simulink model "im_inv_sensorless_ctrl_model"  (R2026a)
settings: Solver=ode1  StopTime=simlength  FixedStep=tc  MaxStep=tc  EnableMultiTasking=on
values from neighbouring files (symbols this model uses):
  cp = 2    [im_param_calc_3.m]
  Ibez = Inom*sqrt(2)    [im_param_calc_3.m]
  Lm = Ls - Lds    [im_param_calc_3.m]
  Lr = Lm + Ldr    [im_param_calc_3.m]
  Ls = Vnom/sqrt(3)/I0/(2*pi*fnom)    [im_param_calc_3.m]
  Rr = Rr+deltaRr    (= 0.00099)    [im_param_calc_3.m]
  Rs = PhaseResistance    (= 0.009)    [im_param_calc_3.m]
undefined symbols (not defined in the file or in its folder): Adrso_im, alpha_norm, beta_norm, Crso_im, CTRPIFF_CLIP_RELEASE, dead_time, DiscIntNeverNeededParam, emf_fb_p, emf_p, fi_rot_ref_norm, fPWM_INV, gamma_norm, iq_lim, Jm_model, kg, ki_inv_d, ki_inv_q, ki_w, kp_inv_d, kp_inv_q, kp_w, kw, Ldrso_im, Lm_norm, Lr_norm, Ls_norm, magnitude, Omega_r_bez, Omega_s_bez, Rs_norm, sigma_norm, simlength, tc, Tcontrol_INV, timeRamp, Tload, ts_afe, ts_inv, uf_omega_ref, uf_uq_ref, wref
libraries: nesl_utility x64, fl_lib x49, simulink x2, im_uvw_2_lib x1, threephase_inductor_lib x1, cstblocks_lti x1
(part 3 of 4)

== system im_inv_sensorless_ctrl_model/inverter//ctrl/im_ctrl/rotor_speed_observer/pi ==
  u_ref : Inport
  u : Inport  Port=2
  1/Ti : Gain  Gain=kp  SaturateOnIntegerOverflow=on  OutDataTypeStr=Inherit: Same as input  ParamDataTypeStr=Inherit: Same as input
  Saturation : Saturate  UpperLimit=lim_up  LowerLimit=lim_down
  Sum1 : Sum  Inputs=+++  SaturateOnIntegerOverflow=on
  Sum2 : Sum  Inputs=-+  SaturateOnIntegerOverflow=on
  Sum3 : Sum  Inputs=-+  SaturateOnIntegerOverflow=on
  Unit Delay4 : UnitDelay  SampleTime=-1
  kp : Gain  Gain=ki  SaturateOnIntegerOverflow=on  OutDataTypeStr=Inherit: Same as input  ParamDataTypeStr=Inherit: Same as input
  y : Outport
  wires:
  1/Ti/1 -> Sum1/1, Sum3/1
  kp/1 -> Sum1/2
  Sum3/1 -> Unit Delay4/1
  Unit Delay4/1 -> Sum1/3
  u_ref/1 -> Sum2/2
  u/1 -> Sum2/1
  Sum2/1 -> kp/1, 1/Ti/1
  Sum1/1 -> Saturation/1
  Saturation/1 -> Sum3/2, y/1

== system im_inv_sensorless_ctrl_model/inverter//ctrl/im_ctrl/rotor_speed_observer/voltage_flux_estimator ==
  Gain : Gain
  Gain1 : Gain
  Trigonometric Function : Trigonometry  Operator=cos
  Trigonometric Function1 : Trigonometry
  Zero-Order Hold{,1..3} (4 alike) : ZeroOrderHold  SampleTime=ts_inv
  flux_observers_from_voltage_model : Scope  NumInputPorts=2
      settings: ActiveDisplayYMinimum=-0.67163437881991128  ActiveDisplayYMaximum=0.85448846422944114  DataLoggingVariableName=ScopeData4
  psi_alpha_hat : Subsystem
  psi_beta_hat : Subsystem
  tag scope: psi_r_alpha_vhat_mod1=global, psi_r_beta_vhat_mod1=global, psi_r_m_alpha=global, psi_r_m_beta=global
  wires:
  Zero-Order Hold3/1 -> psi_beta_hat/2(ibeta)
  psi_alpha_hat/1(psi_r_alpha_hat) -> [psi_r_alpha_vhat_mod1]
  [is_alpha_pu_mod1] -> Zero-Order Hold2/1
  [uctrl_alpha_mod1] -> Zero-Order Hold/1
  [is_beta_pu_mod1] -> Zero-Order Hold3/1
  psi_beta_hat/1(psi_r_beta_hat) -> [psi_r_beta_vhat_mod1]
  [uctrl_beta_mod1] -> Zero-Order Hold1/1
  Zero-Order Hold2/1 -> psi_alpha_hat/2(ialpha)
  Zero-Order Hold/1 -> psi_alpha_hat/1(ualpha)
  Zero-Order Hold1/1 -> psi_beta_hat/1(ubeta)
  [theta_s_mod1] -> Trigonometric Function/1, Trigonometric Function1/1
  Trigonometric Function/1 -> Gain/1
  Trigonometric Function1/1 -> Gain1/1
  Gain1/1 -> [psi_r_m_beta]
  Gain/1 -> [psi_r_m_alpha]
  [psi_r_alpha_vhat_mod1] -> flux_observers_from_voltage_model/1
  [psi_r_beta_vhat_mod1] -> flux_observers_from_voltage_model/2

== system im_inv_sensorless_ctrl_model/inverter//ctrl/inverter/inverter/sv_pwm ==
  ab : Inport
  enable : Inport  Port=2
  pwm_phase : Inport  Port=3
  -1<x<1 : Saturate  UpperLimit=1  LowerLimit=-1
  Bus Selector : BusSelector  OutputSignals=da,db,dc
  C Caller : CCaller  FunctionName=sv_pwm_process_simulink  PortSpecificationStruct="%)30     .    V @   8    (     @         %    \"     4    !     0         %  0 \"0    $    _    07)G3F%M90  4&]R=$YA;64 4V-O<&4     26YD97@     5'EP90      4VEZ90      27-';&]B86P   X    P    !@    @    $          4    (     0    ,    !         !   P!O=70 #@   #     &    \"     0         !0    @    !     P    $         $  # &]U=  .    .     8    (    !          %    \"     $    &     0         0   ...(+2669 chars)"  SampleTime=ts_inv
  Constant : Constant  Value=ts_inv
  Data Type Conversion1 : DataTypeConversion  OutDataTypeStr=double  SaturateOnIntegerOverflow=off  RndMeth=Floor
  Data Type Conversion15 : DataTypeConversion  OutDataTypeStr=single  SaturateOnIntegerOverflow=off  RndMeth=Floor
  Data Type Conversion16 : DataTypeConversion  OutDataTypeStr=single  SaturateOnIntegerOverflow=off  RndMeth=Floor
  Data Type Conversion17 : DataTypeConversion  OutDataTypeStr=uint32  SaturateOnIntegerOverflow=off  RndMeth=Floor
  Data Type Conversion18 : DataTypeConversion  OutDataTypeStr=single  SaturateOnIntegerOverflow=off  RndMeth=Floor
  Data Type Conversion2 : DataTypeConversion  OutDataTypeStr=double  SaturateOnIntegerOverflow=off  RndMeth=Floor
  Data Type Conversion3 : DataTypeConversion  OutDataTypeStr=double  SaturateOnIntegerOverflow=off  RndMeth=Floor
  Demux : Demux  Outputs=2
  Gain : Gain  Gain=sqrt(3)/2
  Zero-Order Hold{,1..3} (4 alike) : ZeroOrderHold  SampleTime=ts_inv
  modulator1 : Subsystem
  cmd_gates : Outport
  wires:
  Demux/2 -> Data Type Conversion15/1
  ab/1 -> -1<x<1/1
  Data Type Conversion3/1 -> modulator1/3(w)  "dw"
  Bus Selector/2 -> Data Type Conversion2/1  "<db>"
  C Caller/1 -> Bus Selector/1  "out"
  Data Type Conversion17/1 -> Zero-Order Hold3/1
  Data Type Conversion15/1 -> Zero-Order Hold1/1
  Data Type Conversion2/1 -> modulator1/2(v)  "dv"
  enable/1 -> Data Type Conversion17/1
  Bus Selector/3 -> Data Type Conversion3/1  "<dc>"
  Data Type Conversion18/1 -> Zero-Order Hold/1
  Bus Selector/1 -> Data Type Conversion1/1  "<da>"
  Constant/1 -> Data Type Conversion16/1
  Data Type Conversion16/1 -> Zero-Order Hold2/1
  Zero-Order Hold/1 -> C Caller/1
  Data Type Conversion1/1 -> modulator1/1(u)  "du"
  Demux/1 -> Data Type Conversion18/1
  pwm_phase/1 -> modulator1/4(phase)
  modulator1/1(cmd_gates) -> cmd_gates/1
  Zero-Order Hold1/1 -> C Caller/2
  Zero-Order Hold2/1 -> C Caller/3
  Zero-Order Hold3/1 -> C Caller/4
  -1<x<1/1 -> Gain/1
  Gain/1 -> Demux/1

== system im_inv_sensorless_ctrl_model/inverter//ctrl/inverter/inverter/switch_1 ==
  Diode : fl_lib/Electrical/Electrical Elements/Diode  Vf=Vgamma V  Ron=Ron Ohm  Goff=1e-8 1/Ohm  i_specify=off  i_priority=None  i=0 A  i_nominal_specify=off  i_nominal_value=1  i_nominal_unit=A  v_specify=off  v_priority=None  v=0 V  v_nominal_specify=off  v_nominal_value=1  v_nominal_unit=V
  Switch : fl_lib/Electrical/Electrical Elements/Switch  R_closed=Ron Ohm  G_open=1e-8 1/Ohm  Threshold=7.5  i_specify=off  i_priority=None  i=0 A  i_nominal_specify=off  i_nominal_value=1  i_nominal_unit=A  v_specify=off  v_priority=None  v=0 V  v_nominal_specify=off  v_nominal_value=1  v_nominal_unit=V
  G : PMIOPort  Side=Left
  C : PMIOPort  Port=2  Side=Left
  E : PMIOPort  Port=3  Side=Right
  connections:
  Diode/LConn1 -- E/RConn1 -- Switch/LConn1
  Switch/RConn1 -- G/RConn1
  Diode/RConn1 -- C/RConn1 -- Switch/RConn2

== system im_inv_sensorless_ctrl_model/inverter//ctrl/inverter/inverter/switch_2 ==
  Diode : fl_lib/Electrical/Electrical Elements/Diode  Vf=Vgamma V  Ron=Ron Ohm  Goff=1e-8 1/Ohm  i_specify=off  i_priority=None  i=0 A  i_nominal_specify=off  i_nominal_value=1  i_nominal_unit=A  v_specify=off  v_priority=None  v=0 V  v_nominal_specify=off  v_nominal_value=1  v_nominal_unit=V
  Switch : fl_lib/Electrical/Electrical Elements/Switch  R_closed=Ron Ohm  G_open=1e-8 1/Ohm  Threshold=7.5  i_specify=off  i_priority=None  i=0 A  i_nominal_specify=off  i_nominal_value=1  i_nominal_unit=A  v_specify=off  v_priority=None  v=0 V  v_nominal_specify=off  v_nominal_value=1  v_nominal_unit=V
  G : PMIOPort  Side=Left
  C : PMIOPort  Port=2  Side=Left
  E : PMIOPort  Port=3  Side=Right
  connections:
  Switch/RConn2 -- C/RConn1 -- Diode/RConn1
  Switch/RConn1 -- G/RConn1
  Switch/LConn1 -- E/RConn1 -- Diode/LConn1

== system im_inv_sensorless_ctrl_model/inverter//ctrl/inverter/inverter/switch_3 ==
  Diode : fl_lib/Electrical/Electrical Elements/Diode  Vf=Vgamma V  Ron=Ron Ohm  Goff=1e-8 1/Ohm  i_specify=off  i_priority=None  i=0 A  i_nominal_specify=off  i_nominal_value=1  i_nominal_unit=A  v_specify=off  v_priority=None  v=0 V  v_nominal_specify=off  v_nominal_value=1  v_nominal_unit=V
  Switch : fl_lib/Electrical/Electrical Elements/Switch  R_closed=Ron Ohm  G_open=1e-8 1/Ohm  Threshold=7.5  i_specify=off  i_priority=None  i=0 A  i_nominal_specify=off  i_nominal_value=1  i_nominal_unit=A  v_specify=off  v_priority=None  v=0 V  v_nominal_specify=off  v_nominal_value=1  v_nominal_unit=V
  G : PMIOPort  Side=Left
  C : PMIOPort  Port=2  Side=Left
  E : PMIOPort  Port=3  Side=Right
  connections:
  Diode/LConn1 -- E/RConn1 -- Switch/LConn1
  Switch/RConn1 -- G/RConn1
  Diode/RConn1 -- C/RConn1 -- Switch/RConn2

== system im_inv_sensorless_ctrl_model/inverter//ctrl/inverter/inverter/switch_4 ==
  Diode : fl_lib/Electrical/Electrical Elements/Diode  Vf=Vgamma V  Ron=Ron Ohm  Goff=1e-8 1/Ohm  i_specify=off  i_priority=None  i=0 A  i_nominal_specify=off  i_nominal_value=1  i_nominal_unit=A  v_specify=off  v_priority=None  v=0 V  v_nominal_specify=off  v_nominal_value=1  v_nominal_unit=V
  Switch : fl_lib/Electrical/Electrical Elements/Switch  R_closed=Ron Ohm  G_open=1e-8 1/Ohm  Threshold=7.5  i_specify=off  i_priority=None  i=0 A  i_nominal_specify=off  i_nominal_value=1  i_nominal_unit=A  v_specify=off  v_priority=None  v=0 V  v_nominal_specify=off  v_nominal_value=1  v_nominal_unit=V
  G : PMIOPort  Side=Left
  C : PMIOPort  Port=2  Side=Left
  E : PMIOPort  Port=3  Side=Right
  connections:
  Switch/RConn2 -- C/RConn1 -- Diode/RConn1
  Switch/RConn1 -- G/RConn1
  Switch/LConn1 -- E/RConn1 -- Diode/LConn1

== system im_inv_sensorless_ctrl_model/inverter//ctrl/inverter/inverter/switch_5 ==
  Diode : fl_lib/Electrical/Electrical Elements/Diode  Vf=Vgamma V  Ron=Ron Ohm  Goff=1e-8 1/Ohm  i_specify=off  i_priority=None  i=0 A  i_nominal_specify=off  i_nominal_value=1  i_nominal_unit=A  v_specify=off  v_priority=None  v=0 V  v_nominal_specify=off  v_nominal_value=1  v_nominal_unit=V
  Switch : fl_lib/Electrical/Electrical Elements/Switch  R_closed=Ron Ohm  G_open=1e-8 1/Ohm  Threshold=7.5  i_specify=off  i_priority=None  i=0 A  i_nominal_specify=off  i_nominal_value=1  i_nominal_unit=A  v_specify=off  v_priority=None  v=0 V  v_nominal_specify=off  v_nominal_value=1  v_nominal_unit=V
  G : PMIOPort  Side=Left
  C : PMIOPort  Port=2  Side=Left
  E : PMIOPort  Port=3  Side=Right
  connections:
  Diode/LConn1 -- E/RConn1 -- Switch/LConn1
  Switch/RConn1 -- G/RConn1
  Diode/RConn1 -- C/RConn1 -- Switch/RConn2

== system im_inv_sensorless_ctrl_model/inverter//ctrl/inverter/inverter/switch_6 ==
  Diode : fl_lib/Electrical/Electrical Elements/Diode  Vf=Vgamma V  Ron=Ron Ohm  Goff=1e-8 1/Ohm  i_specify=off  i_priority=None  i=0 A  i_nominal_specify=off  i_nominal_value=1  i_nominal_unit=A  v_specify=off  v_priority=None  v=0 V  v_nominal_specify=off  v_nominal_value=1  v_nominal_unit=V
  Switch : fl_lib/Electrical/Electrical Elements/Switch  R_closed=Ron Ohm  G_open=1e-8 1/Ohm  Threshold=7.5  i_specify=off  i_priority=None  i=0 A  i_nominal_specify=off  i_nominal_value=1  i_nominal_unit=A  v_specify=off  v_priority=None  v=0 V  v_nominal_specify=off  v_nominal_value=1  v_nominal_unit=V
  G : PMIOPort  Side=Left
  C : PMIOPort  Port=2  Side=Left
  E : PMIOPort  Port=3  Side=Right
  connections:
  Switch/RConn2 -- C/RConn1 -- Diode/RConn1
  Switch/RConn1 -- G/RConn1
  Switch/LConn1 -- E/RConn1 -- Diode/LConn1

== system im_inv_sensorless_ctrl_model/inverter//ctrl/inverter/inverter/three phase pwm ==
  ab : Inport
  enable : Inport  Port=2
  pwm_phase : Inport  Port=3
  Constant : Constant  Value=sqrt(3)/2
  Demux1 : Demux  Outputs=2
  Gain1 : Gain  Gain=1/sqrt(3)
  Gain2 : Gain  Gain=1/sqrt(3)
  Gain3 : Gain  Gain=1/sqrt(3)
  Sum : Sum  Inputs=|+-
  Sum1 : Sum  Inputs=|+-
  Sum2 : Sum  Inputs=|+-
  Sum3 : Sum  Inputs=|++
  Sum4 : Sum  Inputs=|++
  Sum5 : Sum  Inputs=|++
  Third harmonic injecting : Subsystem
  modulator : Subsystem
  uvw2alphabeta1 : MATLAB Function  TreatAsAtomicUnit=on  SystemSampleTime=ts_inv
  cmd_gates : Outport
  wires:
  uvw2alphabeta1/3(w) -> Third harmonic injecting/3(m3), Sum2/1  "wr"
  uvw2alphabeta1/2(v) -> Sum1/1, Third harmonic injecting/2(m2)  "vr"
  uvw2alphabeta1/1(u) -> Sum/1, Third harmonic injecting/1(m1)  "ur"
  Third harmonic injecting/1(trn) -> Sum2/2, Sum/2, Sum1/2
  Demux1/2 -> uvw2alphabeta1/2(beta)
  Demux1/1 -> uvw2alphabeta1/1(alpha)
  ab/1 -> Demux1/1
  Sum/1 -> Sum3/1
  Sum3/1 -> Gain3/1
  Sum1/1 -> Sum4/1
  Sum2/1 -> Sum5/1
  Constant/1 -> Sum3/2, Sum4/2, Sum5/2
  Gain3/1 -> modulator/1(u)
  Sum4/1 -> Gain1/1
  Sum5/1 -> Gain2/1
  Gain1/1 -> modulator/2(v)
  Gain2/1 -> modulator/3(w)
  pwm_phase/1 -> modulator/4(phase)
  modulator/1(cmd_gates) -> cmd_gates/1

== system im_inv_sensorless_ctrl_model/inverter//ctrl/inverter/inverter/three phase pwm1 ==
  ab : Inport
  vdc : Inport  Port=2
  Bus Creator : BusCreator  Inputs=2
  Bus Creator1 : BusCreator  Inputs=2
  Bus Creator2 : BusCreator  Inputs=2
  Bus Creator3 : BusCreator  Inputs=3
  Demux1 : Demux  Outputs=2
  Divide : Product  Inputs=/*
  Divide1 : Product  Inputs=/*
  Divide2 : Product  Inputs=/*
  Gain6 : Gain  Gain=1/sqrt(3)*2
  Gain7 : Gain  Gain=1/sqrt(3)*2
  Gain8 : Gain  Gain=1/sqrt(3)*2
  PWM generator 1 : Subsystem  mask{f=fPWM_INV, ph=0, m_up=1, m_low=-1, dead_time=0}
      mask prompts: f "Frequency"; ph "Phase"; m_up "Max Input Modulation Value"; m_low "Min Input Modulation Value"; dead_time "Dead Time"
  PWM generator 2 : Subsystem  mask{f=fPWM_INV, ph=0, m_up=1, m_low=-1, dead_time=0}
      mask prompts: f "Frequency"; ph "Phase"; m_up "Max Input Modulation Value"; m_low "Min Input Modulation Value"; dead_time "Dead Time"
  PWM generator 3 : Subsystem  mask{f=fPWM_INV, ph=0, m_up=1, m_low=-1, dead_time=0}
      mask prompts: f "Frequency"; ph "Phase"; m_up "Max Input Modulation Value"; m_low "Min Input Modulation Value"; dead_time "Dead Time"
  Sum : Sum  Inputs=|+-
  Sum1 : Sum  Inputs=|+-
  Sum2 : Sum  Inputs=|+-
  Third harmonic injecting : Subsystem
  uvw2alphabeta1 : MATLAB Function  TreatAsAtomicUnit=on  SystemSampleTime=Tcontrol_INV
  duties : Outport
  wires:
  ab/1 -> Demux1/1
  Demux1/1 -> uvw2alphabeta1/1(alpha)
  Demux1/2 -> uvw2alphabeta1/2(beta)
  Third harmonic injecting/1(thind_H) -> Sum1/2, Sum/2, Sum2/2
  uvw2alphabeta1/1(u) -> Third harmonic injecting/1(m1), Sum/1  "ur"
  uvw2alphabeta1/2(v) -> Third harmonic injecting/2(m2), Sum1/1  "vr"
  uvw2alphabeta1/3(w) -> Sum2/1, Third harmonic injecting/3(m3)  "wr"
  vdc/1 -> Divide2/1, Divide1/1, Divide/1
  Sum/1 -> Gain6/1
  Divide/1 -> PWM generator 1/1(m_index)
  Divide2/1 -> PWM generator 3/1(m_index)
  Divide1/1 -> PWM generator 2/1(m_index)
  PWM generator 1/1(m1) -> Bus Creator/1  "gate_cmd_Q1"
  PWM generator 2/1(m1) -> Bus Creator1/1  "gate_cmd_Q3"
  PWM generator 3/1(m1) -> Bus Creator2/1  "gate_cmd_Q5"
  Bus Creator3/1 -> duties/1
  PWM generator 1/2(m2) -> Bus Creator/2  "gate_cmd_Q2"
  PWM generator 2/2(m2) -> Bus Creator1/2  "gate_cmd_Q4"
  PWM generator 3/2(m2) -> Bus Creator2/2  "gate_cmd_Q6"
  Bus Creator1/1 -> Bus Creator3/2  "gate_cmd_leg_v"
  Bus Creator/1 -> Bus Creator3/1  "gate_cmd_leg_u"
  Bus Creator2/1 -> Bus Creator3/3  "gate_cmd_leg_w"
  Gain6/1 -> Divide/2
  Sum1/1 -> Gain7/1
  Sum2/1 -> Gain8/1
  Gain7/1 -> Divide1/2
  Gain8/1 -> Divide2/2

== system im_inv_sensorless_ctrl_model/inverter//ctrl/im_ctrl/im_control/current control/bounder1 ==
  md : Inport
  k_sat : Inport  Port=2
  m : Inport  Port=3
  Constant : Constant
  Constant1 : Constant  Value=0
  Divide : Product
  Switch : Switch  Threshold=sqrt(3)/2  SaturateOnIntegerOverflow=off  InputSameDT=off
  Switch1 : Switch  Threshold=1 %sqrt(3)/2  SaturateOnIntegerOverflow=off  InputSameDT=off
  md_sat : Outport  VectorParamsAs1DForOutWhenUnconnected=off
  clip : Outport  Port=2  VectorParamsAs1DForOutWhenUnconnected=off
  wires:
  md/1 -> Switch1/3, Divide/2
  k_sat/1 -> Divide/1
  Divide/1 -> Switch1/1
  Switch1/1 -> md_sat/1
  Switch/1 -> clip/1
  m/1 -> Switch/2, Switch1/2
  Constant/1 -> Switch/1
  Constant1/1 -> Switch/3

== system im_inv_sensorless_ctrl_model/inverter//ctrl/im_ctrl/im_control/current control/bounder2 ==
  m : Inport
  k_sat : Inport  Port=2
  mq : Inport  Port=3
  Constant : Constant
  Constant1 : Constant  Value=0
  Divide : Product
  Switch : Switch  Threshold=sqrt(3)/2  SaturateOnIntegerOverflow=off  InputSameDT=off
  Switch1 : Switch  Threshold=1 %sqrt(3)/2  SaturateOnIntegerOverflow=off  InputSameDT=off
  mq_sat : Outport  VectorParamsAs1DForOutWhenUnconnected=off
  clip : Outport  Port=2  VectorParamsAs1DForOutWhenUnconnected=off
  wires:
  Constant1/1 -> Switch/3
  Constant/1 -> Switch/1
  m/1 -> Switch1/2, Switch/2
  Switch/1 -> clip/1
  Switch1/1 -> mq_sat/1
  Divide/1 -> Switch1/1
  k_sat/1 -> Divide/1
  mq/1 -> Divide/2, Switch1/3

== system im_inv_sensorless_ctrl_model/inverter//ctrl/im_ctrl/im_control/current control/pi-ctrl-x ==
  id_tilde : Inport
  clip : Inport  Port=2
  1/Ti : Gain  Gain=kp_inv_d  SaturateOnIntegerOverflow=on  OutDataTypeStr=Inherit: Same as input  ParamDataTypeStr=Inherit: Same as input
  Constant : Constant  Value=0
  Sum2 : Sum  Inputs=+-  SaturateOnIntegerOverflow=on
  Sum4 : Sum  SaturateOnIntegerOverflow=on
  Sum5 : Sum  SaturateOnIntegerOverflow=on
  Switch1 : Switch  Threshold=0.5  SaturateOnIntegerOverflow=off  InputSameDT=off
  Switch2 : Switch  Threshold=0.5  SaturateOnIntegerOverflow=off  InputSameDT=off
  Unit Delay1 : UnitDelay  SampleTime=ts_inv
  Unit Delay2 : UnitDelay  SampleTime=ts_inv
  kp1 : Gain  Gain=CTRPIFF_CLIP_RELEASE*ts_inv  SaturateOnIntegerOverflow=on  OutDataTypeStr=Inherit: Same as input  ParamDataTypeStr=Inherit: Same as input
  kp2 : Gain  Gain=ki_inv_d*ts_inv  SaturateOnIntegerOverflow=on  OutDataTypeStr=Inherit: Same as input  ParamDataTypeStr=Inherit: Same as input
  Vds_out : Outport  VectorParamsAs1DForOutWhenUnconnected=off
  wires:
  id_tilde/1 -> kp2/1, 1/Ti/1
  Sum5/1 -> Vds_out/1
  Switch1/1 -> Unit Delay2/1
  Sum4/1 -> Sum5/2, Switch1/3
  kp1/1 -> Sum2/2
  Sum2/1 -> Switch1/1
  Unit Delay2/1 -> Sum4/2, kp1/1, Sum2/1
  1/Ti/1 -> Sum5/1
  Switch2/1 -> Sum4/1
  kp2/1 -> Switch2/3
  clip/1 -> Unit Delay1/1
  [clip] -> Switch2/2
  [clip] -> Switch1/2
  Constant/1 -> Switch2/1
  Unit Delay1/1 -> [clip]

== system im_inv_sensorless_ctrl_model/inverter//ctrl/im_ctrl/im_control/current control/pi-ctrl-y ==
  iq_tilde : Inport
  clip : Inport  Port=2
  1/Ti : Gain  Gain=kp_inv_q  SaturateOnIntegerOverflow=on  OutDataTypeStr=Inherit: Same as input  ParamDataTypeStr=Inherit: Same as input
  Constant : Constant  Value=0
  Sum2 : Sum  Inputs=+-  SaturateOnIntegerOverflow=on
  Sum4 : Sum  SaturateOnIntegerOverflow=on
  Sum5 : Sum  SaturateOnIntegerOverflow=on
  Switch1 : Switch  Threshold=0.5  SaturateOnIntegerOverflow=off  InputSameDT=off
  Switch2 : Switch  Threshold=0.5  SaturateOnIntegerOverflow=off  InputSameDT=off
  Unit Delay1 : UnitDelay  SampleTime=ts_inv
  Unit Delay2 : UnitDelay  SampleTime=ts_inv
  kp1 : Gain  Gain=CTRPIFF_CLIP_RELEASE*ts_inv  SaturateOnIntegerOverflow=on  OutDataTypeStr=Inherit: Same as input  ParamDataTypeStr=Inherit: Same as input
  kp2 : Gain  Gain=ki_inv_q*ts_inv  SaturateOnIntegerOverflow=on  OutDataTypeStr=Inherit: Same as input  ParamDataTypeStr=Inherit: Same as input
  Vqs_out : Outport  VectorParamsAs1DForOutWhenUnconnected=off
  wires:
  Constant/1 -> Switch2/1
  [clip] -> Switch1/2
  [clip] -> Switch2/2
  clip/1 -> Unit Delay1/1
  kp2/1 -> Switch2/3
  Switch2/1 -> Sum4/1
  1/Ti/1 -> Sum5/1
  Unit Delay2/1 -> Sum2/1, kp1/1, Sum4/2
  Sum2/1 -> Switch1/1
  kp1/1 -> Sum2/2
  Sum4/1 -> Sum5/2, Switch1/3
  Switch1/1 -> Unit Delay2/1
  Sum5/1 -> Vqs_out/1
  iq_tilde/1 -> 1/Ti/1, kp2/1
  Unit Delay1/1 -> [clip]

== system im_inv_sensorless_ctrl_model/inverter//ctrl/im_ctrl/im_control/current control/switch ==
  clip 1 : Inport
  clip 2 : Inport  Port=2
  Constant4 : Constant
  Constant5 : Constant  Value=0
  Sum1 : Sum  SaturateOnIntegerOverflow=on
  Switch : Switch  Threshold=0.5  SaturateOnIntegerOverflow=off  InputSameDT=off
  clip : Outport  VectorParamsAs1DForOutWhenUnconnected=off
  wires:
  Constant5/1 -> Switch/3
  Switch/1 -> clip/1
  Constant4/1 -> Switch/1
  Sum1/1 -> Switch/2
  clip 1/1 -> Sum1/1
  clip 2/1 -> Sum1/2

== system im_inv_sensorless_ctrl_model/inverter//ctrl/im_ctrl/im_control/current control/vector lenght ==
  md : Inport
  mq : Inport  Port=2
  1/Ti3 : Gain  Gain=sqrt(3)/2  SaturateOnIntegerOverflow=on  OutDataTypeStr=Inherit: Same as input  ParamDataTypeStr=Inherit: Same as input
  Math Function : Math  Operator=magnitude^2  SignedPower=on
  Math Function1 : Math  Operator=magnitude^2  SignedPower=on
  Math Function2 : Math  Operator=reciprocal  SignedPower=on
  Sqrt : Sqrt
  Sum5 : Sum  SaturateOnIntegerOverflow=on
  k_sat : Outport  VectorParamsAs1DForOutWhenUnconnected=off
  m : Outport  Port=2  VectorParamsAs1DForOutWhenUnconnected=off
  wires:
  Sqrt/1 -> m/1, Math Function2/1
  mq/1 -> Math Function1/1
  Math Function1/1 -> Sum5/2
  Math Function/1 -> Sum5/1
  Sum5/1 -> Sqrt/1
  Math Function2/1 -> k_sat/1
  md/1 -> Math Function/1

== system im_inv_sensorless_ctrl_model/inverter//ctrl/im_ctrl/im_control/data_analysis/double_integrator_observer_1 ==
  theta : Inport
  Gain : Gain  Gain=kw
  Gain1 : Gain  Gain=kg
  Gain2 : Gain  Gain=Omega_s_bez
  Gain3 : Gain  Gain=1/Omega_s_bez
  Gain5 : Gain  Gain=ts_inv
  Sum : Sum  Inputs=-+|
  Sum1 : Sum  Inputs=|++
  Sum2 : Sum  Inputs=|++
  Sum8 : Sum  Inputs=++|
  Unit Delay1 : UnitDelay  InitialCondition=pi  SampleTime=ts_inv
  Unit Delay2 : UnitDelay  SampleTime=ts_inv
  bounder1 : MATLAB Function  TreatAsAtomicUnit=on  SystemSampleTime=ts_inv
  bounder2 : MATLAB Function  TreatAsAtomicUnit=on  SystemSampleTime=ts_inv
  omega_pu_hat : Outport  VectorParamsAs1DForOutWhenUnconnected=off
  wires:
  Gain1/1 -> Sum2/1
  theta/1 -> Sum/2  "theta_bemf"
  Sum8/1 -> Unit Delay1/1
  Unit Delay1/1 -> bounder2/1(u)
  Sum1/1 -> Unit Delay2/1
  Gain/1 -> Gain3/1
  Unit Delay2/1 -> omega_pu_hat/1, Sum1/2, Gain5/1
  Sum2/1 -> Sum8/2
  bounder2/1(y) -> Sum2/2, Sum/1  "theta_hat"
  bounder1/1(y) -> Gain1/1, Gain/1
  Gain2/1 -> Sum8/1
  Gain3/1 -> Sum1/1
  Gain5/1 -> Gain2/1
  Sum/1 -> bounder1/1(u)

== system im_inv_sensorless_ctrl_model/inverter//ctrl/im_ctrl/im_control/data_analysis/double_integrator_observer_2 ==
  theta : Inport
  Gain : Gain  Gain=kw
  Gain1 : Gain  Gain=kg
  Gain2 : Gain  Gain=Omega_s_bez
  Gain3 : Gain  Gain=1/Omega_s_bez
  Gain5 : Gain  Gain=ts_inv
  Sum : Sum  Inputs=-+|
  Sum1 : Sum  Inputs=|++
  Sum2 : Sum  Inputs=|++
  Sum8 : Sum  Inputs=++|
  Unit Delay1 : UnitDelay  InitialCondition=pi  SampleTime=ts_inv
  Unit Delay2 : UnitDelay  SampleTime=ts_inv
  bounder1 : MATLAB Function  TreatAsAtomicUnit=on  SystemSampleTime=ts_inv
  bounder2 : MATLAB Function  TreatAsAtomicUnit=on  SystemSampleTime=ts_inv
  omega_pu_hat : Outport  VectorParamsAs1DForOutWhenUnconnected=off
  wires:
  Sum/1 -> bounder1/1(u)
  Gain5/1 -> Gain2/1
  Gain3/1 -> Sum1/1
  Gain2/1 -> Sum8/1
  bounder1/1(y) -> Gain/1, Gain1/1
  bounder2/1(y) -> Sum/1, Sum2/2  "theta_hat"
  Sum2/1 -> Sum8/2
  Unit Delay2/1 -> Gain5/1, Sum1/2, omega_pu_hat/1
  Gain/1 -> Gain3/1
  Sum1/1 -> Unit Delay2/1
  Unit Delay1/1 -> bounder2/1(u)
  Sum8/1 -> Unit Delay1/1
  theta/1 -> Sum/2  "theta_bemf"
  Gain1/1 -> Sum2/1

== system im_inv_sensorless_ctrl_model/inverter//ctrl/im_ctrl/im_control/data_analysis/double_integrator_observer_3 ==
  theta : Inport
  Gain : Gain  Gain=kw
  Gain1 : Gain  Gain=kg
  Gain2 : Gain  Gain=Omega_s_bez
  Gain3 : Gain  Gain=1/Omega_s_bez
  Gain5 : Gain  Gain=ts_inv
  Sum : Sum  Inputs=-+|
  Sum1 : Sum  Inputs=|++
  Sum2 : Sum  Inputs=|++
  Sum8 : Sum  Inputs=++|
  Unit Delay1 : UnitDelay  InitialCondition=pi  SampleTime=ts_inv
  Unit Delay2 : UnitDelay  SampleTime=ts_inv
  bounder1 : MATLAB Function  TreatAsAtomicUnit=on  SystemSampleTime=ts_inv
  bounder2 : MATLAB Function  TreatAsAtomicUnit=on  SystemSampleTime=ts_inv
  omega_pu_hat : Outport  VectorParamsAs1DForOutWhenUnconnected=off
  wires:
  Gain1/1 -> Sum2/1
  theta/1 -> Sum/2  "theta_bemf"
  Sum8/1 -> Unit Delay1/1
  Unit Delay1/1 -> bounder2/1(u)
  Sum1/1 -> Unit Delay2/1
  Gain/1 -> Gain3/1
  Unit Delay2/1 -> omega_pu_hat/1, Sum1/2, Gain5/1
  Sum2/1 -> Sum8/2
  bounder2/1(y) -> Sum2/2, Sum/1  "theta_hat"
  bounder1/1(y) -> Gain1/1, Gain/1
  Gain2/1 -> Sum8/1
  Gain3/1 -> Sum1/1
  Gain5/1 -> Gain2/1
  Sum/1 -> bounder1/1(u)

== system im_inv_sensorless_ctrl_model/inverter//ctrl/im_ctrl/im_control/flux_estimator/alphabeta2dq ==
  alpha : Inport
  beta : Inport  Port=2
  phase : Inport  Port=3
  Gain : Gain
  Gain1 : Gain
  Product{,1..3} (4 alike) : Product  RndMeth=Zero
  Sum : Sum
  Sum1 : Sum  Inputs=-+
  Trigonometric Function : Trigonometry  Operator=cos
  Trigonometric Function1 : Trigonometry
  d : Outport  VectorParamsAs1DForOutWhenUnconnected=off
  q : Outport  Port=2  VectorParamsAs1DForOutWhenUnconnected=off
  wires:
  [cos] -> Product/1
  alpha/1 -> Product/2, Product2/2
  Product/1 -> Sum/1
  Product1/1 -> Sum/2
  [sin] -> Product1/1
  beta/1 -> Product1/2, Product3/2
  Sum/1 -> Gain/1
  [sin] -> Product2/1
  Product2/1 -> Sum1/1
  Product3/1 -> Sum1/2
  [cos] -> Product3/1
  Sum1/1 -> Gain1/1
  Gain/1 -> d/1
  Gain1/1 -> q/1
  Trigonometric Function1/1 -> [sin]
  Trigonometric Function/1 -> [cos]
  phase/1 -> Trigonometric Function/1, Trigonometric Function1/1

== system im_inv_sensorless_ctrl_model/inverter//ctrl/im_ctrl/im_control/magnetization current reference/pi ==
  psi_r_hat : Inport
  psi_r_ref : Inport  Port=2
  1/Ti : Gain  Gain=2  SaturateOnIntegerOverflow=on  OutDataTypeStr=Inherit: Same as input  ParamDataTypeStr=Inherit: Same as input
  Saturation : Saturate  UpperLimit=0.6*Lm_norm  LowerLimit=0.05*Lm_norm
  Sum1 : Sum  Inputs=+++  SaturateOnIntegerOverflow=on
  Sum2 : Sum  Inputs=-+  SaturateOnIntegerOverflow=on
  Sum3 : Sum  Inputs=-+  SaturateOnIntegerOverflow=on
  Unit Delay4 : UnitDelay  SampleTime=ts_inv
  kp : Gain  Gain=20*ts_inv  SaturateOnIntegerOverflow=on  OutDataTypeStr=Inherit: Same as input  ParamDataTypeStr=Inherit: Same as input
  psi_s_ref : Outport  VectorParamsAs1DForOutWhenUnconnected=off
  wires:
  1/Ti/1 -> Sum1/1, Sum3/1
  kp/1 -> Sum1/2
  Sum2/1 -> 1/Ti/1, kp/1
  Sum1/1 -> Saturation/1
  Sum3/1 -> Unit Delay4/1
  Unit Delay4/1 -> Sum1/3
  psi_r_ref/1 -> Sum2/2
  psi_r_hat/1 -> Sum2/1
  Saturation/1 -> psi_s_ref/1, Sum3/2

== system im_inv_sensorless_ctrl_model/inverter//ctrl/im_ctrl/im_control/u//f control/uf_phase_generation ==
  Constant1 : Constant  Value=uf_omega_ref
  Gain : Gain  Gain=Omega_s_bez
  Integrator : Integrator
  Zero-Order Hold : ZeroOrderHold  SampleTime=ts_inv
  bounder : MATLAB Function  TreatAsAtomicUnit=on  SystemSampleTime=ts_inv
  uf_electrical_phase : Outport
  wires:
  Gain/1 -> Integrator/1
  Integrator/1 -> Zero-Order Hold/1
  Zero-Order Hold/1 -> bounder/1(u)
  Constant1/1 -> Gain/1
  bounder/1(y) -> uf_electrical_phase/1

== system im_inv_sensorless_ctrl_model/inverter//ctrl/im_ctrl/rotor_speed_observer/current_flux_estimator/alphabeta2dq ==
  alpha : Inport
  beta : Inport  Port=2
  phase : Inport  Port=3
  Gain : Gain
  Gain1 : Gain
  Product{,1..3} (4 alike) : Product  RndMeth=Zero
  Sum : Sum
  Sum1 : Sum  Inputs=-+
  Trigonometric Function : Trigonometry  Operator=cos
  Trigonometric Function1 : Trigonometry
  d : Outport  VectorParamsAs1DForOutWhenUnconnected=off
  q : Outport  Port=2  VectorParamsAs1DForOutWhenUnconnected=off
  wires:
  [cos] -> Product/1
  alpha/1 -> Product/2, Product2/2
  Product/1 -> Sum/1
  Product1/1 -> Sum/2
  [sin] -> Product1/1
  beta/1 -> Product1/2, Product3/2
  Sum/1 -> Gain/1
  [sin] -> Product2/1
  Product2/1 -> Sum1/1
  Product3/1 -> Sum1/2
  [cos] -> Product3/1
  Sum1/1 -> Gain1/1
  Gain/1 -> d/1
  Gain1/1 -> q/1
  Trigonometric Function1/1 -> [sin]
  Trigonometric Function/1 -> [cos]
  phase/1 -> Trigonometric Function/1, Trigonometric Function1/1

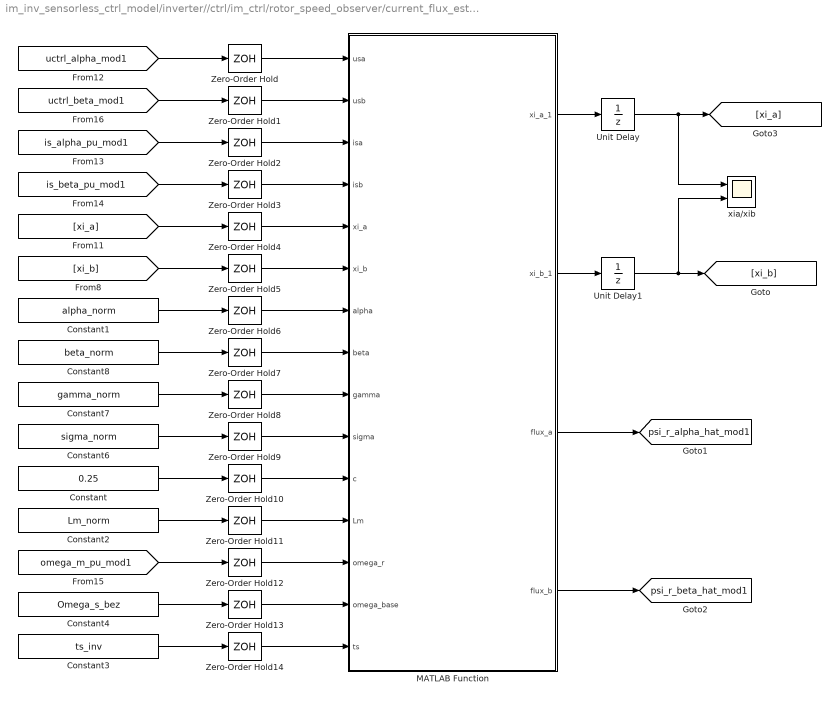
== system im_inv_sensorless_ctrl_model/inverter//ctrl/im_ctrl/rotor_speed_observer/current_flux_estimator/obs_td ==
  Constant : Constant  Value=0.25
  Constant1 : Constant  Value=alpha_norm
  Constant2 : Constant  Value=Lm_norm
  Constant3 : Constant  Value=ts_inv
  Constant4 : Constant  Value=Omega_s_bez
  Constant6 : Constant  Value=sigma_norm
  Constant7 : Constant  Value=gamma_norm
  Constant8 : Constant  Value=beta_norm
  MATLAB Function : MATLAB Function  TreatAsAtomicUnit=on  SystemSampleTime=ts_inv
  Unit Delay : UnitDelay  InitialCondition=fi_rot_ref_norm  SampleTime=ts_inv
  Unit Delay1 : UnitDelay  SampleTime=ts_inv
  Zero-Order Hold{,1..14} (15 alike) : ZeroOrderHold  SampleTime=ts_inv
  xia/xib : Scope  NumInputPorts=2
      settings: ActiveDisplayYMinimum=-0.88025764378851079  ActiveDisplayYMaximum=1.1781452232755658  DataLoggingVariableName=ScopeData11
  tag scope: psi_r_alpha_hat_mod1=global, psi_r_beta_hat_mod1=global
  wires:
  MATLAB Function/1(xi_a_1) -> Unit Delay/1
  Constant6/1 -> Zero-Order Hold9/1
  [xi_b] -> Zero-Order Hold5/1
  MATLAB Function/3(flux_a) -> [psi_r_alpha_hat_mod1]
  Constant2/1 -> Zero-Order Hold11/1
  Constant7/1 -> Zero-Order Hold8/1
  Constant4/1 -> Zero-Order Hold13/1
  MATLAB Function/4(flux_b) -> [psi_r_beta_hat_mod1]
  Unit Delay/1 -> [xi_a], xia/xib/1
  [xi_a] -> Zero-Order Hold4/1
  [is_beta_pu_mod1] -> Zero-Order Hold3/1
  [omega_m_pu_mod1] -> Zero-Order Hold12/1
  MATLAB Function/2(xi_b_1) -> Unit Delay1/1
  [is_alpha_pu_mod1] -> Zero-Order Hold2/1
  Constant8/1 -> Zero-Order Hold7/1
  Constant1/1 -> Zero-Order Hold6/1
  Zero-Order Hold3/1 -> MATLAB Function/4(isb)
  Zero-Order Hold11/1 -> MATLAB Function/12(Lm)
  Zero-Order Hold2/1 -> MATLAB Function/3(isa)
  Zero-Order Hold14/1 -> MATLAB Function/15(ts)
  Zero-Order Hold/1 -> MATLAB Function/1(usa)
  Zero-Order Hold12/1 -> MATLAB Function/13(omega_r)
  Zero-Order Hold5/1 -> MATLAB Function/6(xi_b)
  Zero-Order Hold9/1 -> MATLAB Function/10(sigma)
  Zero-Order Hold6/1 -> MATLAB Function/7(alpha)
  Zero-Order Hold8/1 -> MATLAB Function/9(gamma)
  Zero-Order Hold13/1 -> MATLAB Function/14(omega_base)
  Zero-Order Hold7/1 -> MATLAB Function/8(beta)
  Zero-Order Hold10/1 -> MATLAB Function/11(c)
  Zero-Order Hold4/1 -> MATLAB Function/5(xi_a)
  Zero-Order Hold1/1 -> MATLAB Function/2(usb)
  Constant3/1 -> Zero-Order Hold14/1
  Unit Delay1/1 -> [xi_b], xia/xib/2
  Constant/1 -> Zero-Order Hold10/1
  [uctrl_alpha_mod1] -> Zero-Order Hold/1
  [uctrl_beta_mod1] -> Zero-Order Hold1/1

== system im_inv_sensorless_ctrl_model/inverter//ctrl/im_ctrl/rotor_speed_observer/voltage_flux_estimator/psi_alpha_hat ==
  ualpha : Inport
  ialpha : Inport  Port=2
  Gain1 : Gain  Gain=Rs_norm
  Gain2 : Gain  Gain=emf_fb_p
  Gain3 : Gain  Gain=emf_p
  Gain4 : Gain  Gain=Omega_s_bez
  Gain5 : Gain  Gain=sigma_norm*Ls_norm
  Gain7 : Gain  Gain=ts_inv
  Gain8 : Gain  Gain=Lr_norm/Lm_norm
  Sum : Sum  Inputs=|+-
  Sum1 : Sum  Inputs=|+-
  Sum2 : Sum  Inputs=++-  SaturateOnIntegerOverflow=on
  Sum3 : Sum  Inputs=|++
  Sum4 : Sum  Inputs=+-  SaturateOnIntegerOverflow=on
  Unit Delay1 : UnitDelay  SampleTime=ts_inv
  Unit Delay2 : UnitDelay  SampleTime=ts_inv
  Unit Delay3 : UnitDelay  SampleTime=ts_inv
  psi_r_alpha_hat : Outport  VectorParamsAs1DForOutWhenUnconnected=off
  wires:
  [psi_r_m_alpha] -> Sum1/1
  [psi_r_alpha_vhat_mod1] -> Sum1/2
  Gain4/1 -> Gain7/1
  Sum2/1 -> Gain8/1
  Gain3/1 -> Sum2/3
  ialpha/1 -> Gain5/1, Gain1/1
  Gain1/1 -> Sum/2
  Sum/1 -> Sum2/2
  Gain5/1 -> Unit Delay3/1
  Unit Delay1/1 -> Sum4/1, Gain3/1, Sum3/2
  Sum3/1 -> Unit Delay1/1
  Sum4/1 -> Unit Delay2/1
  Sum1/1 -> Gain2/1
  Gain2/1 -> Sum2/1
  Gain7/1 -> Sum3/1
  ualpha/1 -> Sum/1
  Unit Delay2/1 -> psi_r_alpha_hat/1
  Unit Delay3/1 -> Sum4/2
  Gain8/1 -> Gain4/1

== system im_inv_sensorless_ctrl_model/inverter//ctrl/im_ctrl/rotor_speed_observer/voltage_flux_estimator/psi_beta_hat ==
  ubeta : Inport
  ibeta : Inport  Port=2
  Gain1 : Gain  Gain=Rs_norm
  Gain2 : Gain  Gain=emf_fb_p
  Gain3 : Gain  Gain=emf_p
  Gain4 : Gain  Gain=Omega_s_bez
  Gain5 : Gain  Gain=sigma_norm*Ls_norm
  Gain7 : Gain  Gain=ts_inv
  Gain8 : Gain  Gain=Lr_norm/Lm_norm
  Sum : Sum  Inputs=|+-
  Sum1 : Sum  Inputs=|+-
  Sum2 : Sum  Inputs=++-  SaturateOnIntegerOverflow=on
  Sum3 : Sum  Inputs=|++
  Sum4 : Sum  Inputs=+-  SaturateOnIntegerOverflow=on
  Unit Delay1 : UnitDelay  SampleTime=ts_inv
  Unit Delay2 : UnitDelay  SampleTime=ts_inv
  Unit Delay3 : UnitDelay  SampleTime=ts_inv
  psi_r_beta_hat : Outport  VectorParamsAs1DForOutWhenUnconnected=off
  wires:
  Gain5/1 -> Unit Delay3/1
  Sum/1 -> Sum2/2
  Gain1/1 -> Sum/2
  ibeta/1 -> Gain5/1, Gain1/1
  Gain3/1 -> Sum2/3
  Sum2/1 -> Gain8/1
  Gain4/1 -> Gain7/1
  Sum1/1 -> Gain2/1
  [psi_r_beta_vhat_mod1] -> Sum1/2
  [psi_r_m_beta] -> Sum1/1
  Unit Delay1/1 -> Gain3/1, Sum4/1, Sum3/2
  Sum3/1 -> Unit Delay1/1
  Sum4/1 -> Unit Delay2/1
  Gain2/1 -> Sum2/1
  Gain7/1 -> Sum3/1
  ubeta/1 -> Sum/1
  Unit Delay2/1 -> psi_r_beta_hat/1
  Unit Delay3/1 -> Sum4/2
  Gain8/1 -> Gain4/1

== system im_inv_sensorless_ctrl_model/inverter//ctrl/inverter/inverter/sv_pwm/modulator1 ==
  u : Inport
  v : Inport  Port=2
  w : Inport  Port=3
  phase : Inport  Port=4
  Bus Creator3 : BusCreator  Inputs=6
  PWM generator 1 : Subsystem  mask{f=fPWM_INV, m_up=0.98, m_low=0.02, dead_time=dead_time, pos_cmd_gate=15, neg_cmd_gate=-10, polarity=-1}
      mask prompts: f "Frequency (Hz)"; m_up "Max Input Modulation Value"; m_low "Min Input Modulation Value"; dead_time "Dead Time (s)"; pos_cmd_gate "Positive Gate Voltage (V)"; neg_cmd_gate "Negative Gate Voltage (V)"; polarity "Polarity (pu)"
  PWM generator 2 : Subsystem  mask{f=fPWM_INV, m_up=0.98, m_low=0.02, dead_time=dead_time, pos_cmd_gate=15, neg_cmd_gate=-10, polarity=-1}
      mask prompts: f "Frequency (Hz)"; m_up "Max Input Modulation Value"; m_low "Min Input Modulation Value"; dead_time "Dead Time (s)"; pos_cmd_gate "Positive Gate Voltage (V)"; neg_cmd_gate "Negative Gate Voltage (V)"; polarity "Polarity (pu)"
  PWM generator 3 : Subsystem  mask{f=fPWM_INV, m_up=0.98, m_low=0.02, dead_time=dead_time, pos_cmd_gate=15, neg_cmd_gate=-10, polarity=-1}
      mask prompts: f "Frequency (Hz)"; m_up "Max Input Modulation Value"; m_low "Min Input Modulation Value"; dead_time "Dead Time (s)"; pos_cmd_gate "Positive Gate Voltage (V)"; neg_cmd_gate "Negative Gate Voltage (V)"; polarity "Polarity (pu)"
  cmd_gates : Outport
  wires:
  u/1 -> PWM generator 1/1(m_index)
  w/1 -> PWM generator 3/1(m_index)
  v/1 -> PWM generator 2/1(m_index)
  phase/1 -> PWM generator 3/2(phase), PWM generator 2/2(phase), PWM generator 1/2(phase)
  PWM generator 1/2(m2) -> Bus Creator3/2  "gate_cmd_Q2"
  PWM generator 3/1(m1) -> Bus Creator3/5  "gate_cmd_Q5"
  PWM generator 2/1(m1) -> Bus Creator3/3  "gate_cmd_Q3"
  PWM generator 2/2(m2) -> Bus Creator3/4  "gate_cmd_Q4"
  PWM generator 3/2(m2) -> Bus Creator3/6  "gate_cmd_Q6"
  PWM generator 1/1(m1) -> Bus Creator3/1  "gate_cmd_Q1"
  Bus Creator3/1 -> cmd_gates/1

== system im_inv_sensorless_ctrl_model/inverter//ctrl/inverter/inverter/three phase pwm/Third harmonic injecting ==
  m1 : Inport
  m2 : Inport  Port=2
  m3 : Inport  Port=3
  Gain : Gain  Gain=1/2
  MinMax : MinMax  Function=max  Inputs=3
  MinMax1 : MinMax  Inputs=3
  Sum : Sum  Inputs=|++
  trn : Outport
  wires:
  Gain/1 -> trn/1
  Sum/1 -> Gain/1
  MinMax1/1 -> Sum/2
  MinMax/1 -> Sum/1
  m3/1 -> MinMax/3, MinMax1/3
  m1/1 -> MinMax1/1, MinMax/1
  m2/1 -> MinMax1/2, MinMax/2

== system im_inv_sensorless_ctrl_model/inverter//ctrl/inverter/inverter/three phase pwm/modulator ==
  u : Inport
  v : Inport  Port=2
  w : Inport  Port=3
  phase : Inport  Port=4
  Bus Creator3 : BusCreator  Inputs=6
  PWM generator 1 : Subsystem  mask{f=fPWM_INV, m_up=1, m_low=0, dead_time=0, vg_firing=15}
      mask prompts: f "Frequency"; m_up "Max Input Modulation Value"; m_low "Min Input Modulation Value"; dead_time "Dead Time"; vg_firing "Gate Voltage"
  PWM generator 2 : Subsystem  mask{f=fPWM_INV, m_up=1, m_low=0, dead_time=0, vg_firing=15}
      mask prompts: f "Frequency"; m_up "Max Input Modulation Value"; m_low "Min Input Modulation Value"; dead_time "Dead Time"; vg_firing "Gate Voltage"
  PWM generator 3 : Subsystem  mask{f=fPWM_INV, m_up=1, m_low=0, dead_time=0, vg_firing=15}
      mask prompts: f "Frequency"; m_up "Max Input Modulation Value"; m_low "Min Input Modulation Value"; dead_time "Dead Time"; vg_firing "Gate Voltage"
  cmd_gates : Outport
  wires:
  u/1 -> PWM generator 1/1(m_index)
  w/1 -> PWM generator 3/1(m_index)
  v/1 -> PWM generator 2/1(m_index)
  phase/1 -> PWM generator 3/2(phase), PWM generator 2/2(phase), PWM generator 1/2(phase)
  PWM generator 3/2(m2) -> Bus Creator3/6  "gate_cmd_Q6"
  Bus Creator3/1 -> cmd_gates/1
  PWM generator 2/2(m2) -> Bus Creator3/4  "gate_cmd_Q4"
  PWM generator 1/1(m1) -> Bus Creator3/1  "gate_cmd_Q1"
  PWM generator 3/1(m1) -> Bus Creator3/5  "gate_cmd_Q5"
  PWM generator 1/2(m2) -> Bus Creator3/2  "gate_cmd_Q2"
  PWM generator 2/1(m1) -> Bus Creator3/3  "gate_cmd_Q3"

== system im_inv_sensorless_ctrl_model/inverter//ctrl/inverter/inverter/three phase pwm1/PWM generator 1 ==
  m_index : Inport
  Constant : Constant  Value=dead_time*f*2
  Data Type Conversion1 : DataTypeConversion
  Data Type Conversion2 : DataTypeConversion
  Gain : Gain  Gain=1/(pi/2)
  Gain1 : Gain  Gain=sqrt(3)/2
  Hit Crossing : HitCross  ShowOutputPort=off
  Hit Crossing1 : HitCross  ShowOutputPort=off
  Relational Operator1 : RelationalOperator  Operator=<=  InputSameDT=off
  Relational Operator2 : RelationalOperator  Operator=<=  InputSameDT=off
  Saturation1 : Saturate  UpperLimit=m_up  LowerLimit=m_low
  Sine Wave : Sin  Frequency=f*2*pi  Phase=-pi/2+ph  SampleTime=0
  Sum : Sum  Inputs=|++  SaturateOnIntegerOverflow=on
  Sum1 : Sum  Inputs=-+|  SaturateOnIntegerOverflow=on
  Trigonometric Function1 : Trigonometry  Operator=asin
  m1 : Outport
  m2 : Outport  Port=2
  wires:
  Relational Operator1/1 -> Data Type Conversion1/1
  m_index/1 -> Saturation1/1
  Data Type Conversion1/1 -> Hit Crossing/1, m2/1
  Relational Operator2/1 -> Data Type Conversion2/1
  Data Type Conversion2/1 -> Hit Crossing1/1, m1/1
  Constant/1 -> Sum/2, Sum1/1
  Saturation1/1 -> Sum/1, Sum1/2
  Sum/1 -> Relational Operator1/1
  Sum1/1 -> Relational Operator2/2
  Sine Wave/1 -> Trigonometric Function1/1
  Trigonometric Function1/1 -> Gain/1
  Gain/1 -> Gain1/1
  Gain1/1 -> Relational Operator1/2, Relational Operator2/1

== system im_inv_sensorless_ctrl_model/inverter//ctrl/inverter/inverter/three phase pwm1/PWM generator 2 ==
  m_index : Inport
  Constant : Constant  Value=dead_time*f*2
  Data Type Conversion1 : DataTypeConversion
  Data Type Conversion2 : DataTypeConversion
  Gain : Gain  Gain=1/(pi/2)
  Gain1 : Gain  Gain=sqrt(3)/2
  Hit Crossing : HitCross  ShowOutputPort=off
  Hit Crossing1 : HitCross  ShowOutputPort=off
  Relational Operator1 : RelationalOperator  Operator=<=  InputSameDT=off
  Relational Operator2 : RelationalOperator  Operator=<=  InputSameDT=off
  Saturation1 : Saturate  UpperLimit=m_up  LowerLimit=m_low
  Sine Wave : Sin  Frequency=f*2*pi  Phase=-pi/2+ph  SampleTime=0
  Sum : Sum  Inputs=|++  SaturateOnIntegerOverflow=on
  Sum1 : Sum  Inputs=-+|  SaturateOnIntegerOverflow=on
  Trigonometric Function1 : Trigonometry  Operator=asin
  m1 : Outport
  m2 : Outport  Port=2
  wires:
  Gain1/1 -> Relational Operator2/1, Relational Operator1/2
  Gain/1 -> Gain1/1
  Trigonometric Function1/1 -> Gain/1
  Sine Wave/1 -> Trigonometric Function1/1
  Sum1/1 -> Relational Operator2/2
  Sum/1 -> Relational Operator1/1
  Saturation1/1 -> Sum1/2, Sum/1
  Constant/1 -> Sum1/1, Sum/2
  Data Type Conversion2/1 -> m1/1, Hit Crossing1/1
  Relational Operator2/1 -> Data Type Conversion2/1
  Data Type Conversion1/1 -> m2/1, Hit Crossing/1
  m_index/1 -> Saturation1/1
  Relational Operator1/1 -> Data Type Conversion1/1

== system im_inv_sensorless_ctrl_model/inverter//ctrl/inverter/inverter/three phase pwm1/PWM generator 3 ==
  m_index : Inport
  Constant : Constant  Value=dead_time*f*2
  Data Type Conversion1 : DataTypeConversion
  Data Type Conversion2 : DataTypeConversion
  Gain : Gain  Gain=1/(pi/2)
  Gain1 : Gain  Gain=sqrt(3)/2
  Hit Crossing : HitCross  ShowOutputPort=off
  Hit Crossing1 : HitCross  ShowOutputPort=off
  Relational Operator1 : RelationalOperator  Operator=<=  InputSameDT=off
  Relational Operator2 : RelationalOperator  Operator=<=  InputSameDT=off
  Saturation1 : Saturate  UpperLimit=m_up  LowerLimit=m_low
  Sine Wave : Sin  Frequency=f*2*pi  Phase=-pi/2+ph  SampleTime=0
  Sum : Sum  Inputs=|++  SaturateOnIntegerOverflow=on
  Sum1 : Sum  Inputs=-+|  SaturateOnIntegerOverflow=on
  Trigonometric Function1 : Trigonometry  Operator=asin
  m1 : Outport
  m2 : Outport  Port=2
  wires:
  Relational Operator1/1 -> Data Type Conversion1/1
  m_index/1 -> Saturation1/1
  Data Type Conversion1/1 -> Hit Crossing/1, m2/1
  Relational Operator2/1 -> Data Type Conversion2/1
  Data Type Conversion2/1 -> Hit Crossing1/1, m1/1
  Constant/1 -> Sum/2, Sum1/1
  Saturation1/1 -> Sum/1, Sum1/2
  Sum/1 -> Relational Operator1/1
  Sum1/1 -> Relational Operator2/2
  Sine Wave/1 -> Trigonometric Function1/1
  Trigonometric Function1/1 -> Gain/1
  Gain/1 -> Gain1/1
  Gain1/1 -> Relational Operator1/2, Relational Operator2/1

== system im_inv_sensorless_ctrl_model/inverter//ctrl/inverter/inverter/three phase pwm1/Third harmonic injecting ==
  m1 : Inport
  m2 : Inport  Port=2
  m3 : Inport  Port=3
  Gain : Gain  Gain=1/2
  MinMax : MinMax  Function=max  Inputs=3
  MinMax1 : MinMax  Inputs=3
  Sum : Sum  Inputs=|++
  thind_H : Outport
  wires:
  m2/1 -> MinMax/2, MinMax1/2
  m1/1 -> MinMax/1, MinMax1/1
  m3/1 -> MinMax/3, MinMax1/3
  MinMax/1 -> Sum/1
  MinMax1/1 -> Sum/2
  Sum/1 -> Gain/1
  Gain/1 -> thind_H/1

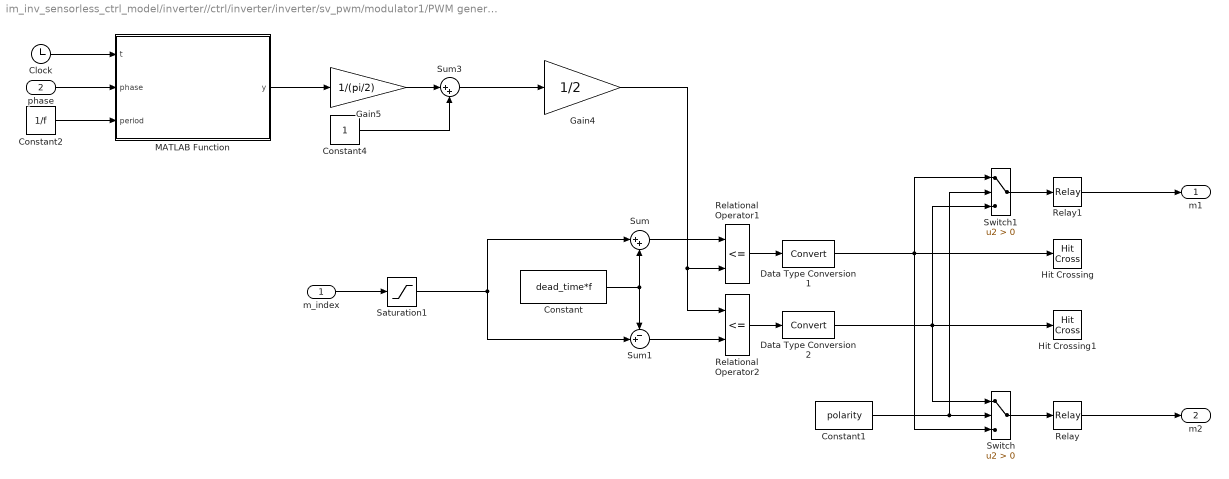
== system im_inv_sensorless_ctrl_model/inverter//ctrl/inverter/inverter/sv_pwm/modulator1/PWM generator 1 ==
  m_index : Inport
  phase : Inport  Port=2
  Clock : Clock
  Constant : Constant  Value=dead_time*f
  Constant1 : Constant  Value=polarity
  Constant2 : Constant  Value=1/f
  Constant4 : Constant
  Data Type Conversion1 : DataTypeConversion
  Data Type Conversion2 : DataTypeConversion
  Gain4 : Gain  Gain=1/2
  Gain5 : Gain  Gain=1/(pi/2)
  Hit Crossing : HitCross  ShowOutputPort=off
  Hit Crossing1 : HitCross  ShowOutputPort=off
  MATLAB Function : MATLAB Function  TreatAsAtomicUnit=on
  Relational Operator1 : RelationalOperator  Operator=<=  InputSameDT=off
  Relational Operator2 : RelationalOperator  Operator=<=  InputSameDT=off
  Relay : Relay  OnOutputValue=pos_cmd_gate  OffOutputValue=neg_cmd_gate
  Relay1 : Relay  OnOutputValue=pos_cmd_gate  OffOutputValue=neg_cmd_gate
  Saturation1 : Saturate  UpperLimit=m_up  LowerLimit=m_low
  Sum : Sum  Inputs=|++  SaturateOnIntegerOverflow=on
  Sum1 : Sum  Inputs=-+|  SaturateOnIntegerOverflow=on
  Sum3 : Sum  Inputs=|++
  Switch : Switch  Criteria=u2 > Threshold  SaturateOnIntegerOverflow=off  InputSameDT=off
  Switch1 : Switch  Criteria=u2 > Threshold  SaturateOnIntegerOverflow=off  InputSameDT=off
  m1 : Outport
  m2 : Outport  Port=2
  wires:
  Relational Operator1/1 -> Data Type Conversion1/1
  m_index/1 -> Saturation1/1
  Relational Operator2/1 -> Data Type Conversion2/1
  Data Type Conversion2/1 -> Switch/1, Switch1/3, Hit Crossing1/1
  Constant/1 -> Sum/2, Sum1/1
  Saturation1/1 -> Sum/1, Sum1/2
  Sum/1 -> Relational Operator1/1
  Sum1/1 -> Relational Operator2/2
  Gain4/1 -> Relational Operator2/1, Relational Operator1/2
  Data Type Conversion1/1 -> Hit Crossing/1, Switch/3, Switch1/1
  Switch/1 -> Relay/1
  Clock/1 -> MATLAB Function/1(t)
  Constant2/1 -> MATLAB Function/3(period)
  phase/1 -> MATLAB Function/2(phase)
  MATLAB Function/1(y) -> Gain5/1
  Gain5/1 -> Sum3/1
  Sum3/1 -> Gain4/1
  Constant4/1 -> Sum3/2
  Relay/1 -> m2/1
  Constant1/1 -> Switch1/2, Switch/2
  Switch1/1 -> Relay1/1
  Relay1/1 -> m1/1

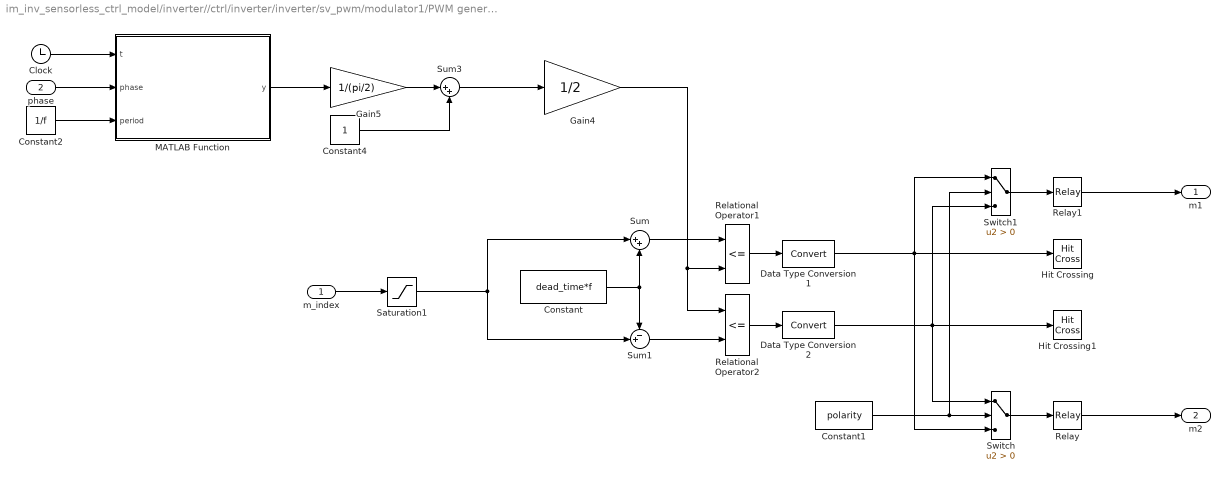
== system im_inv_sensorless_ctrl_model/inverter//ctrl/inverter/inverter/sv_pwm/modulator1/PWM generator 2 ==
  m_index : Inport
  phase : Inport  Port=2
  Clock : Clock
  Constant : Constant  Value=dead_time*f
  Constant1 : Constant  Value=polarity
  Constant2 : Constant  Value=1/f
  Constant4 : Constant
  Data Type Conversion1 : DataTypeConversion
  Data Type Conversion2 : DataTypeConversion
  Gain4 : Gain  Gain=1/2
  Gain5 : Gain  Gain=1/(pi/2)
  Hit Crossing : HitCross  ShowOutputPort=off
  Hit Crossing1 : HitCross  ShowOutputPort=off
  MATLAB Function : MATLAB Function  TreatAsAtomicUnit=on
  Relational Operator1 : RelationalOperator  Operator=<=  InputSameDT=off
  Relational Operator2 : RelationalOperator  Operator=<=  InputSameDT=off
  Relay : Relay  OnOutputValue=pos_cmd_gate  OffOutputValue=neg_cmd_gate
  Relay1 : Relay  OnOutputValue=pos_cmd_gate  OffOutputValue=neg_cmd_gate
  Saturation1 : Saturate  UpperLimit=m_up  LowerLimit=m_low
  Sum : Sum  Inputs=|++  SaturateOnIntegerOverflow=on
  Sum1 : Sum  Inputs=-+|  SaturateOnIntegerOverflow=on
  Sum3 : Sum  Inputs=|++
  Switch : Switch  Criteria=u2 > Threshold  SaturateOnIntegerOverflow=off  InputSameDT=off
  Switch1 : Switch  Criteria=u2 > Threshold  SaturateOnIntegerOverflow=off  InputSameDT=off
  m1 : Outport
  m2 : Outport  Port=2
  wires:
  Relay1/1 -> m1/1
  Switch1/1 -> Relay1/1
  Constant1/1 -> Switch/2, Switch1/2
  Relay/1 -> m2/1
  Constant4/1 -> Sum3/2
  Sum3/1 -> Gain4/1
  Gain5/1 -> Sum3/1
  MATLAB Function/1(y) -> Gain5/1
  phase/1 -> MATLAB Function/2(phase)
  Constant2/1 -> MATLAB Function/3(period)
  Clock/1 -> MATLAB Function/1(t)
  Switch/1 -> Relay/1
  Data Type Conversion1/1 -> Switch1/1, Switch/3, Hit Crossing/1
  Gain4/1 -> Relational Operator1/2, Relational Operator2/1
  Sum1/1 -> Relational Operator2/2
  Sum/1 -> Relational Operator1/1
  Saturation1/1 -> Sum1/2, Sum/1
  Constant/1 -> Sum1/1, Sum/2
  Data Type Conversion2/1 -> Hit Crossing1/1, Switch1/3, Switch/1
  Relational Operator2/1 -> Data Type Conversion2/1
  m_index/1 -> Saturation1/1
  Relational Operator1/1 -> Data Type Conversion1/1
